simulink model "hopper_6dof_NED_v3_fluid_integration"  (R2026a)
settings: Solver=FixedStepAuto  StopTime=30  FixedStep=1e-3  RelTol=1e-5
InitFcn:
  | load('FuelPropsData.mat');
undefined symbols (not defined in the file): bp, cg_init, dcg_dMfu_table, dcg_dMox_table, dI_dMfu_table, dI_dMox_table, ENGINE, engine_cg, engine_mass, fu_masses, g, IN, K1flat, K2grid, MoI_init, mount_cg, OUT, ox_masses, pressureLevels, r_leg_1, r_leg_2, r_leg_3, r_leg_4, tank_r, TANKS, Target_Trajectory_full, tbl1, tbl2, tgrid, unom, uwndTable, VEH, vwndTable
libraries: fl_lib x43, nesl_utility x31, matrix_library x18, SimscapeFluids_lib x13, simulink_extras x7, slpidlib x7, simulink x7, dspindex x3, sl_discontinuities x2, aerolibanim x1, commrandsrc3 x1, aerolibutil x1
(part 2 of 7)

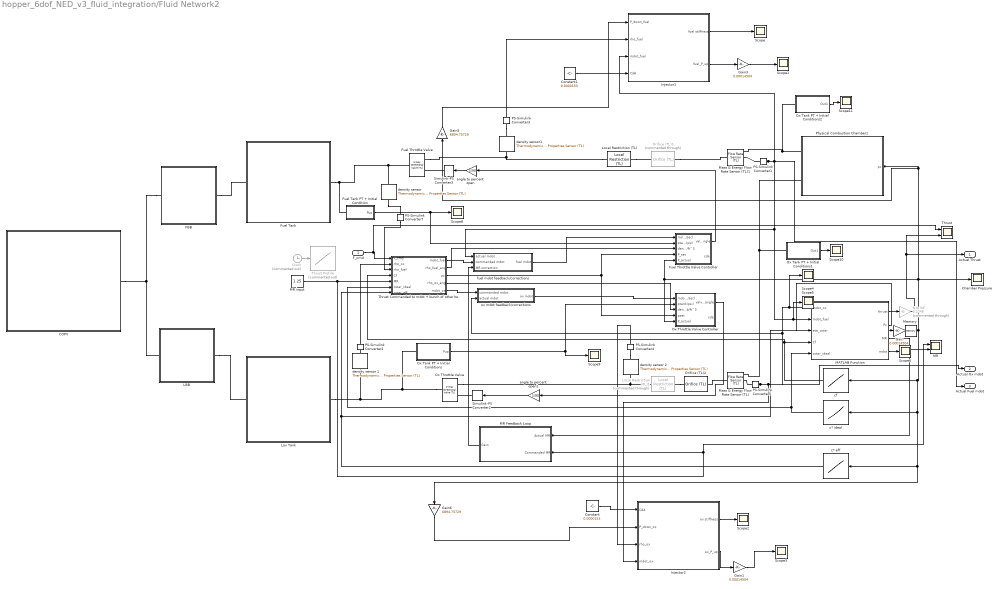
== system hopper_6dof_NED_v3_fluid_integration/Fluid Network2 ==
  F_cmd : Inport
  COPV : Subsystem
  Chamber Pressure : Scope
      settings: ActiveDisplayYMinimum=24.4768520913143  ActiveDisplayYMaximum=276.14956071215624  DataLoggingVariableName=ScopeData22
  Clock : Clock  Commented=on
  Constant : Constant  Value=0.0000153
  Constant1 : Constant  Value=0.0000153
  FBB : Subsystem
  Fuel Tank : Subsystem
  Fuel Tank PT + Initial Condition : Subsystem
  Fuel Throttle Valve : SimscapeFluids_lib/Thermal Liquid/Valves & Orifices/Directional Control Valves/2-Way Directional Valve (TL)  valve_spec=fluids.thermal_liquid.valves.directional_control_valves.enum.ValveSpec.Table1DAreaOpening  S_max=1 m  del_S_max=5e-3 m  area_max=1e-4 m^2  area_leak=1e-10 m^2  del_S_TLU=[0 0.3 0.4 0.5 0.6 0.7 0.8 0.9 1.0] m  valve_area_TLU=[1e-9 1.7065e-07 1.0239e-06 3.5836e-06 7.8498e-06 1.4164e-05 2.3038e-05 3.4812e-05 5.0000e-05] m^2  del_S_flow_TLU=[0, .002, .004, .007, .017] m  p_diff_TLU=[.3, .5, .7] MPa  vol_flow_TLU=1e-3 * [1.7e-05, 2e-05, 2.6e-05; .0035, .0045, .0053; .7, .9, 1.06; 1.96, 2.5, 3; 6, 7.7, 9.13] m^3/s  mdot_TLU=[1.7e-05, 2e-05, 2.6e-05; .0035, .0045, .0053; .7, .9, 1.06; 1.96, 2.5, 3; 6, 7.7, 9.13] kg/s  T_ref_in=293.15 K  p_ref_in=0.101325 MPa  Cd=1  Re_c=150  smoothing_factor=0.01  pressure_recovery=false  area=0.01 m^2
  Fuel Throttle Valve Controller : Subsystem
  Gain : Gain  Gain=0.00014504
  Gain1 : Gain  Gain=0.00014504
  Gain3 : Gain  Gain=0.00014504
  Gain5 : Gain  Gain=6894.75729
  Gain6 : Gain  Gain=6894.75729
  Injector1 : Subsystem
  Injector2 : Subsystem
  LBB : Subsystem
  Local Restriction (TL) : fl_lib/Thermal Liquid/Elements/Local Restriction (TL)  restriction_type=foundation.enum.restriction_type.fixed  restriction_area=0.0000153 m^2  min_area=1e-10 m^2  max_area=0.005 m^2  area=0.000153 m^2  Cd=1  Re_c=150  pressure_recovery=true
  Local Restriction (TL)1 : fl_lib/Thermal Liquid/Elements/Local Restriction (TL)  Commented=through  restriction_type=foundation.enum.restriction_type.fixed  restriction_area=0.0000153 m^2  min_area=1e-10 m^2  max_area=0.005 m^2  area=0.000153 m^2  Cd=1  Re_c=150  pressure_recovery=true
  Lox Tank : Subsystem
  MATLAB Function : MATLAB Function  TreatAsAtomicUnit=on
  MR : Scope  NumInputPorts=2
      settings: ActiveDisplayYMinimum=0.081947452963374467  ActiveDisplayYMaximum=2.5817499803566988
  MR Feedback Loop : Subsystem
  MR input : Constant  Value=1.25
  Mass & Energy Flow Rate Sensor (TL) : fl_lib/Thermal Liquid/Sensors/Flow Rate Sensor (TL)  mass_flow_measure=true  volumetric_flow_measure=false  energy_flow_measure=true
  Mass & Energy Flow Rate Sensor (TL)1 : fl_lib/Thermal Liquid/Sensors/Flow Rate Sensor (TL)  mass_flow_measure=true  volumetric_flow_measure=false  energy_flow_measure=true
  Memory : Memory  InitialCondition=300
  N to lbf : Gain  Commented=through  Gain=0.2248
  Orifice (TL)1 : SimscapeFluids_lib/Thermal Liquid/Valves & Orifices/Orifice (TL)  Commented=through  orifice_type=foundation.enum.constant_variable.constant  constant_orifice_spec=fluids.thermal_liquid.valves.enum.ConstantOrificeSpec.Area  variable_orifice_spec=fluids.thermal_liquid.valves.enum.orifice_spec.linear  orifice_area_constant=0.0000153 m^2  p_diff_TLU_constant=[-4, -3, -2, -1, -.5, 0, .5, 1, 2, 3, 4] MPa  vol_flow_TLU_constant=[-2.44, -2.12, -1.68, -1.22, -.84, 0, .85, 1.21, 1.7, 2.09, 2.41] .* 1e-3 m^3/s  mdot_TLU_constant=[-2.44, -2.12, -1.68, -1.22, -.84, 0, .85, 1.21, 1.7, 2.09, 2.41] kg/s  S_min=0 m  del_S=5e-3 m  open_orientation=fluids.thermal_liquid.valves.enum.orifice_orientation.positive  area_max=1e-4 m^2  area_leak=1e-10 m^2  S_TLU=[0, .002, .004, .007, .017] m  orifice_area_TLU=[1e-09, 2.0352e-07, 4.0736e-05, .00011438, .00034356] m^2  Cd=1  Re_c=150  smoothing_factor=0.01  pressure_recovery=false  S_flow_TLU=[0, .002, .004, .007, .017] m  p_diff_TLU=[.3, .5, .7] MPa  vol_flow_TLU=1e-3 * [1.7e-05, 2e-05, 2.6e-05; .0035, .0045, .0053; .7, .9, 1.06; 1.96, 2.5, 3; 6, 7.7, 9.13] m^3/s  mdot_TLU=[1.7e-05, 2e-05, 2.6e-05; .0035, .0045, .0053; .7, .9, 1.06; 1.96, 2.5, 3; 6, 7.7, 9.13] kg/s  T_ref_in=293.15 K  p_ref_in=0.101325 MPa  area=0.01 m^2
  Orifice (TL)2 : SimscapeFluids_lib/Thermal Liquid/Valves & Orifices/Orifice (TL)  orifice_type=foundation.enum.constant_variable.constant  constant_orifice_spec=fluids.thermal_liquid.valves.enum.ConstantOrificeSpec.Area  variable_orifice_spec=fluids.thermal_liquid.valves.enum.orifice_spec.linear  orifice_area_constant=0.0000153 m^2  p_diff_TLU_constant=[-4, -3, -2, -1, -.5, 0, .5, 1, 2, 3, 4] MPa  vol_flow_TLU_constant=[-2.44, -2.12, -1.68, -1.22, -.84, 0, .85, 1.21, 1.7, 2.09, 2.41] .* 1e-3 m^3/s  mdot_TLU_constant=[-2.44, -2.12, -1.68, -1.22, -.84, 0, .85, 1.21, 1.7, 2.09, 2.41] kg/s  S_min=0 m  del_S=5e-3 m  open_orientation=fluids.thermal_liquid.valves.enum.orifice_orientation.positive  area_max=1e-4 m^2  area_leak=1e-10 m^2  S_TLU=[0, .002, .004, .007, .017] m  orifice_area_TLU=[1e-09, 2.0352e-07, 4.0736e-05, .00011438, .00034356] m^2  Cd=1  Re_c=150  smoothing_factor=0.01  pressure_recovery=false  S_flow_TLU=[0, .002, .004, .007, .017] m  p_diff_TLU=[.3, .5, .7] MPa  vol_flow_TLU=1e-3 * [1.7e-05, 2e-05, 2.6e-05; .0035, .0045, .0053; .7, .9, 1.06; 1.96, 2.5, 3; 6, 7.7, 9.13] m^3/s  mdot_TLU=[1.7e-05, 2e-05, 2.6e-05; .0035, .0045, .0053; .7, .9, 1.06; 1.96, 2.5, 3; 6, 7.7, 9.13] kg/s  T_ref_in=293.15 K  p_ref_in=0.101325 MPa  area=0.01 m^2
  Ox Tank PT + Initial Conditions : Subsystem
  Ox Tank PT + Initial Conditions1 : Subsystem
  Ox Tank PT + Initial Conditions2 : Subsystem
  Ox Throttle Valve : SimscapeFluids_lib/Thermal Liquid/Valves & Orifices/Directional Control Valves/2-Way Directional Valve (TL)  valve_spec=fluids.thermal_liquid.valves.directional_control_valves.enum.ValveSpec.Table1DAreaOpening  S_max=1 m  del_S_max=5e-3 m  area_max=1e-4 m^2  area_leak=1e-10 m^2  del_S_TLU=[0 0.3 0.4 0.5 0.6 0.7 0.8 0.9 1.0] m  valve_area_TLU=[1e-9 1.7065e-07 1.0239e-06 3.5836e-06 7.8498e-06 1.4164e-05 2.3038e-05 3.4812e-05 5.0000e-05] m^2  del_S_flow_TLU=[0, .002, .004, .007, .017] m  p_diff_TLU=[.3, .5, .7] MPa  vol_flow_TLU=1e-3 * [1.7e-05, 2e-05, 2.6e-05; .0035, .0045, .0053; .7, .9, 1.06; 1.96, 2.5, 3; 6, 7.7, 9.13] m^3/s  mdot_TLU=[1.7e-05, 2e-05, 2.6e-05; .0035, .0045, .0053; .7, .9, 1.06; 1.96, 2.5, 3; 6, 7.7, 9.13] kg/s  T_ref_in=293.15 K  p_ref_in=0.101325 MPa  Cd=1  Re_c=150  smoothing_factor=0.01  pressure_recovery=false  area=0.01 m^2
  Ox Throttle Valve Controller : Subsystem
  PS-Simulink Converter{1..5,7} (6 alike) : nesl_utility/PS-Simulink Converter  PhysicalDomain=network_engine_domain  SubClassName=ps_output  LeftPortType=input  RightPortType=output  PseudoPeriodic=off  Frequencies=[]  VectorFormat=inherit  Unit=inherit  AffineConversion=off
  Physical Combustion Chamber1 : Subsystem
  Scope{,1..6,8..11} (11 alike) : Scope
      Scope settings: ActiveDisplayYMinimum=-0.024254245068718681  ActiveDisplayYMaximum=0.21828827495285463  DataLoggingVariableName=ScopeData40
      Scope1 settings: ActiveDisplayYMinimum=-37.465424615708343  ActiveDisplayYMaximum=337.50135970832162  DataLoggingVariableName=ScopeData42
      Scope10 settings: ActiveDisplayYMinimum=-62.731329785992315  ActiveDisplayYMaximum=586.85713455527571  DataLoggingVariableName=ScopeData51
      Scope11 settings: ActiveDisplayYMinimum=-62.499971643181283  ActiveDisplayYMaximum=562.49999684924239  DataLoggingVariableName=ScopeData52
      Scope2 settings: ActiveDisplayYMinimum=-0.025857157768165939  ActiveDisplayYMaximum=0.4462125176132366  DataLoggingVariableName=ScopeData43
      Scope3 settings: ActiveDisplayYMinimum=-1  ActiveDisplayYMaximum=1  DataLoggingVariableName=ScopeData44
      Scope4 settings: ActiveDisplayYMinimum=-0.071595374751251564  ActiveDisplayYMaximum=0.64519605918641931  DataLoggingVariableName=ScopeData53
      Scope5 settings: ActiveDisplayYMinimum=-0.05515719954820638  ActiveDisplayYMaximum=0.49713967255882957  DataLoggingVariableName=ScopeData54
      Scope6 settings: ActiveDisplayYMinimum=-0.1205205125313115  ActiveDisplayYMaximum=1.086247175831931  DataLoggingVariableName=ScopeData55
      Scope8 settings: ActiveDisplayYMinimum=481.05362935967628  ActiveDisplayYMaximum=536.06057249536832  DataLoggingVariableName=ScopeData49
      Scope9 settings: ActiveDisplayYMinimum=492.10107740407369  ActiveDisplayYMaximum=524.51908611925091  DataLoggingVariableName=ScopeData50
  Simulink-PS Converter2 : nesl_utility/Simulink-PS Converter  PhysicalDomain=network_engine_domain  SubClassName=ps_input  LeftPortType=input  RightPortType=output  PseudoPeriodic=off  Frequencies=[]  NoiseDistribution=none  NoiseParameters=[]  Unit=1  AffineConversion=off  FilteringAndDerivatives=filter  SimscapeFilterOrder=1  InputFilterTimeConstant=0.001  UdotUserProvided=0
  Simulink-PS Converter3 : nesl_utility/Simulink-PS Converter  PhysicalDomain=network_engine_domain  SubClassName=ps_input  LeftPortType=input  RightPortType=output  PseudoPeriodic=off  Frequencies=[]  NoiseDistribution=none  NoiseParameters=[]  Unit=1  AffineConversion=off  FilteringAndDerivatives=filter  SimscapeFilterOrder=1  InputFilterTimeConstant=0.001  UdotUserProvided=0
  Thrust : Scope  NumInputPorts=2
      settings: ActiveDisplayYMinimum=-215.53569406218494  ActiveDisplayYMaximum=1942.1553478833205  DataLoggingVariableName=ScopeData21
  Thrust Commanded to mdot + bunch of other bs : MATLAB Function  TreatAsAtomicUnit=on
  Thrust Profile : Lookup_n-D  Commented=on  NumberOfTableDimensions=1  BreakpointsForDimension1=|  Table=|  InternalRulePriority=Speed  RndMeth=Simplest
      BreakpointsForDimension1=|
      | [0
      | 2.46e-15
      | 4.93e-15
      | 1.31e-14
      | 1.85798e-4
      | 3.71595e-4
      | 1.300583e-3
      | 5.945524e-3
      | 2.917023e-2
      | 1.452937e-1
      | 3.251823e-1
      | 6.176896e-1
      | 1.048884
      | 1.648122
      | 2.452841
      | 3.452841
      | 4.452841
      | 5.452841
      | 6.452841
      | 7.452841
      | 8.452841
      | 9.452841
      | 10.45284
      | 11.45284
      | 12.45284
      | 13.45284
      | 14.45284
      | 15.45284
      | 16.26888
      | 17.26888
      | 18.26888
      | 19.26888
      | 20.26888
      | 21.26888
      | 21.82014
      | 22.37140
      | 23.10183
      | 24.10183
      | 25.10183
      | 26.10183
      | 27.10183
      | 28.10183
      | 29.10183
      | 29.70287]
      Table=|
      | [1115.929794
      | 1115.929794
      | 1115.929794
      | 1115.929794
      | 1116.015031
      | 1116.100248
      | 1116.526042
      | 1118.647732
      | 1129.075722
      | 1176.888468
      | 1237.984070
      | 1309.087819
      | 1365.657208
      | 1382.500173
      | 1347.869214
      | 1276.732855
      | 1209.886660
      | 1007.359221
      | 890.000000
      | 890.000000
      | 890.000000
      | 890.000000
      | 970.372958
      | 1015.368113
      | 1034.720854
      | 1040.888013
      | 1040.596927
      | 896.870767
      | 890.000000
      | 890.000000
      | 890.000000
      | 890.000000
      | 890.000000
      | 890.000000
      | 1074.062231
      | 1213.486737
      | 1218.338865
      | 1172.384789
      | 1114.978943
      | 1066.195681
      | 1030.043331
      | 1004.841448
      | 987.599936
      | 979.912878]
  angle to percent open : Gain  Gain=1/90
  angle to percent open1 : Gain  Gain=1/90
  c* eff : Lookup_n-D  NumberOfTableDimensions=1  BreakpointsForDimension1=[125 295]  Table=[0.8 0.85]  InternalRulePriority=Speed  RndMeth=Simplest
  c* ideal : Lookup_n-D  NumberOfTableDimensions=1  BreakpointsForDimension1=[100 110 120 130 140 150 160 170 180 190 200 210 220 230 240 250 260 270 280 290 300 310 320 330 340 350]  Table=[1492.810749 1492.812678 1492.815823 1492.820080 1492.825344 1492.831574 1492.838703 1492.846662 1492.855462 1492.865052 1492.875406 1492.886504 1492.898325 1492.910854 1492.924078 1492.937982 1492.952558 1492.967791 1492.983688 1493.000184 1493.017345 1493.035113 1493.053494 1493.072480 1493.092063 1493.112237]  InternalRulePriority=Speed  RndMeth=Simplest
  cf : Lookup_n-D  NumberOfTableDimensions=1  BreakpointsForDimension1=[125 295]  Table=[1.42 1.57]  InternalRulePriority=Speed  RndMeth=Simplest
  density sensor : fl_lib/Thermal Liquid/Sensors/Thermodynamic Properties Sensor (TL)  internal_energy=false  density=true  specific_heat=false
  density sensor 1 : fl_lib/Thermal Liquid/Sensors/Thermodynamic Properties Sensor (TL)  internal_energy=false  density=true  specific_heat=false
  density sensor 2 : fl_lib/Thermal Liquid/Sensors/Thermodynamic Properties Sensor (TL)  internal_energy=false  density=true  specific_heat=false
  density sensor1 : fl_lib/Thermal Liquid/Sensors/Thermodynamic Properties Sensor (TL)  internal_energy=false  density=true  specific_heat=false
  fuel mdot feedback/corrections : Subsystem
  ox mdot feedback/corrections : Subsystem
  Actual Thrust : Outport
  Actual Ox mdot : Outport  Port=2
  Actual Fuel mdot : Outport  Port=3
  wires:
  MATLAB Function/4(mdot) -> Scope6/1
  PS-Simulink Converter4/1 -> Injector2/3(rho_ox)
  PS-Simulink Converter3/1 -> Injector1/2(rho_fuel)
  Memory/1 -> Chamber Pressure/1, Fuel Throttle Valve Controller/5(P_actual), Ox Throttle Valve Controller/5(P_actual), Physical Combustion Chamber1/1(pc), Gain5/1, cf/1, c* ideal/1, c* eff/1, Gain6/1
  Gain6/1 -> Injector2/2(P_down_ox)
  Gain5/1 -> Injector1/1(P_down_fuel)
  Gain1/1 -> Scope3/1
  Gain3/1 -> Scope1/1
  Ox Tank PT + Initial Conditions2/1(Out1) -> Scope11/1
  Ox Tank PT + Initial Conditions1/1(Out1) -> Scope10/1
  PS-Simulink Converter7/1 -> Thrust Commanded to mdot + bunch of other bs/3(rho_fuel)
  Constant1/1 -> Injector1/4(CdA)
  Constant/1 -> Injector2/1(CdA)
  Injector2/2(ox_P_up) -> Gain1/1
  Injector2/1(ox stiffness) -> Scope2/1
  Injector1/2(fuel_P_up) -> Gain3/1
  Injector1/1(fuel stiffness) -> Scope/1
  PS-Simulink Converter1/1 -> fuel mdot feedback/corrections/1(actual mdot), MATLAB Function/2(mdot_fuel), Scope5/1, Injector1/3(mdot_fuel), Actual Fuel mdot/1
  PS-Simulink Converter5/1 -> ox mdot feedback/corrections/2(actual mdot), MATLAB Function/1(mdot_ox), Scope4/1, Injector2/4(mdot_ox), Actual Ox mdot/1
  F_cmd/1 -> Thrust Commanded to mdot + bunch of other bs/1(F_cmd), Thrust/1
  cf/1 -> MATLAB Function/4(Cf), Thrust Commanded to mdot + bunch of other bs/4(Cf)
  c* eff/1 -> MATLAB Function/3(eta_cstar), Thrust Commanded to mdot + bunch of other bs/7(cstar_eff)
  PS-Simulink Converter2/1 -> Thrust Commanded to mdot + bunch of other bs/2(rho_ox)
  Thrust Commanded to mdot + bunch of other bs/3(pc) -> Fuel Throttle Valve Controller/4(P_set), Ox Throttle Valve Controller/4(pset)
  MR input/1 -> Thrust Commanded to mdot + bunch of other bs/5(MR), MR/1, MR Feedback Loop/2(Commanded MR)
  MR Feedback Loop/1(Gain) -> fuel mdot feedback/corrections/3(MR correction)
  ox mdot feedback/corrections/1(ox mdot) -> Ox Throttle Valve Controller/1(mdot (lb/sec))
  MATLAB Function/2(Pc) -> Gain/1
  Fuel Throttle Valve Controller/1(valve angle) -> angle to percent open/1
  Gain/1 -> Memory/1
  MATLAB Function/1(thrust) -> N to lbf/1
  Clock/1 -> Thrust Profile/1
  Thrust Commanded to mdot + bunch of other bs/4(rho_ox_eng) -> Ox Throttle Valve Controller/3(density lb/ft^3)
  Thrust Commanded to mdot + bunch of other bs/5(mdot_ox) -> ox mdot feedback/corrections/1(commanded mdot)
  fuel mdot feedback/corrections/1(fuel mdot) -> Fuel Throttle Valve Controller/1(mdot (lb/sec))
  MATLAB Function/3(MR) -> MR/2, MR Feedback Loop/1(Actual MR)
  angle to percent open1/1 -> Simulink-PS Converter2/1
  angle to percent open/1 -> Simulink-PS Converter3/1
  Ox Tank PT + Initial Conditions/1(Pup) -> Ox Throttle Valve Controller/2(ptank(psi)), Scope9/1
  Thrust Commanded to mdot + bunch of other bs/1(mdot_fuel) -> fuel mdot feedback/corrections/2(commanded mdot)
  N to lbf/1 -> Actual Thrust/1, Thrust/2
  Fuel Tank PT + Initial Condition/1(Pup) -> Fuel Throttle Valve Controller/2(ptank(psi)), Scope8/1
  Thrust Commanded to mdot + bunch of other bs/2(rho_fuel_eng) -> Fuel Throttle Valve Controller/3(density lb/ft^3)
  Ox Throttle Valve Controller/1(valve angle) -> angle to percent open1/1
  c* ideal/1 -> Thrust Commanded to mdot + bunch of other bs/6(cstar_ideal), MATLAB Function/5(cstar_ideal)
  connections:
  Local Restriction (TL)1/RConn1 -- Orifice (TL)2/LConn1
  Local Restriction (TL)/RConn1 -- Orifice (TL)1/LConn1
  PS-Simulink Converter4/LConn1 -- density sensor 2/RConn1
  PS-Simulink Converter3/LConn1 -- density sensor1/RConn1
  Orifice (TL)2/RConn1 -- Mass & Energy Flow Rate Sensor (TL)/LConn1
  Orifice (TL)1/RConn1 -- Mass & Energy Flow Rate Sensor (TL)1/LConn1
  Local Restriction (TL)/LConn1 -- density sensor1/LConn1 -- Fuel Throttle Valve/RConn2
  Simulink-PS Converter2/RConn1 -- Ox Throttle Valve/RConn1
  PS-Simulink Converter1/LConn1 -- Mass & Energy Flow Rate Sensor (TL)1/RConn2
  FBB/LConn1 -- LBB/LConn1 -- COPV/RConn1
  Ox Throttle Valve/LConn1 -- Ox Tank PT + Initial Conditions/LConn1 -- density sensor 1/LConn1 -- Lox Tank/RConn1
  density sensor/RConn1 -- PS-Simulink Converter7/LConn1
  Mass & Energy Flow Rate Sensor (TL)/RConn1 -- Physical Combustion Chamber1/RConn2 -- Ox Tank PT + Initial Conditions1/LConn1
  FBB/RConn1 -- Fuel Tank/LConn1
  Ox Tank PT + Initial Conditions2/LConn1 -- Physical Combustion Chamber1/RConn1 -- Mass & Energy Flow Rate Sensor (TL)1/RConn1
  density sensor 2/LConn1 -- Local Restriction (TL)1/LConn1 -- Ox Throttle Valve/RConn2
  PS-Simulink Converter5/LConn1 -- Mass & Energy Flow Rate Sensor (TL)/RConn2
  Simulink-PS Converter3/RConn1 -- Fuel Throttle Valve/RConn1
  Fuel Tank PT + Initial Condition/LConn1 -- density sensor/LConn1 -- Fuel Throttle Valve/LConn1 -- Fuel Tank/RConn1
  LBB/RConn1 -- Lox Tank/LConn1
  density sensor 1/RConn1 -- PS-Simulink Converter2/LConn1

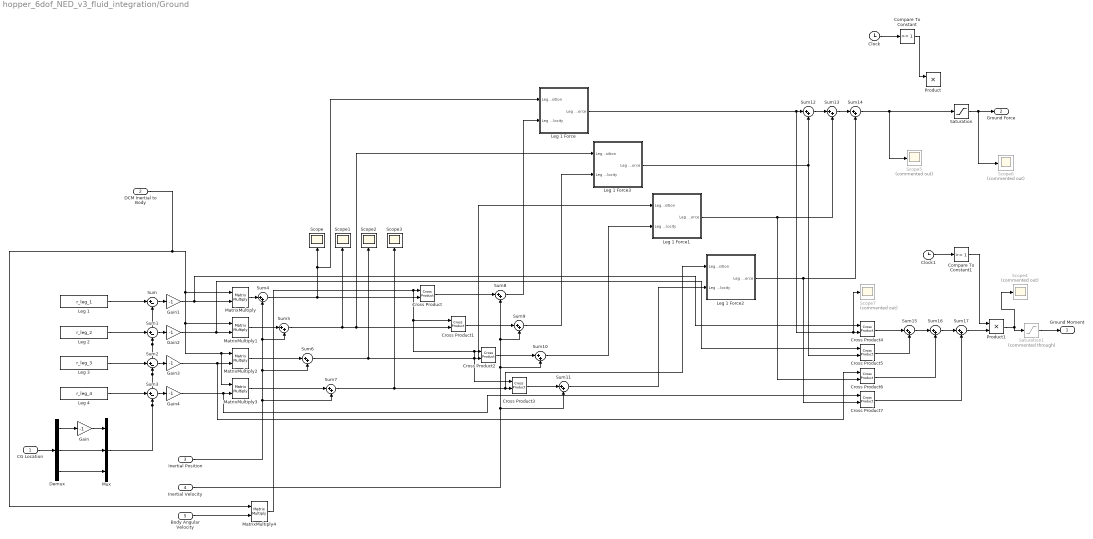
== system hopper_6dof_NED_v3_fluid_integration/Ground  ==
  CG Location : Inport
  DCM Inertial to Body : Inport  Port=2
  Inertial Position : Inport  Port=3
  Inertial Velocity : Inport  Port=4
  Body Angular Velocity : Inport  Port=5
  Clock : Clock
  Clock1 : Clock
  Compare To Constant : simulink/Logic and Bit Operations/Compare To Constant  relop=>=  const=1  OutDataTypeStr=boolean
  Compare To Constant1 : simulink/Logic and Bit Operations/Compare To Constant  relop=>=  const=1  OutDataTypeStr=boolean
  Cross Product{,1..7} (8 alike) : matrix_library/Cross Product
  Demux : Demux  Outputs=3
  Gain{,1..4} (5 alike) : Gain  Gain=-1
  Leg 1 : Constant  Value=r_leg_1
  Leg 1 Force : Subsystem
  Leg 1 Force1 : Subsystem
  Leg 1 Force2 : Subsystem
  Leg 1 Force3 : Subsystem
  Leg 2 : Constant  Value=r_leg_2
  Leg 3 : Constant  Value=r_leg_3
  Leg 4 : Constant  Value=r_leg_4
  MatrixMultiply{,1..4} (5 alike) : Product  Multiplication=Matrix(*)
  Mux : Mux  Inputs=3
  Product : Product
  Product1 : Product
  Saturation : Saturate  UpperLimit=inf  LowerLimit=0
  Saturation1 : Saturate  Commented=through  UpperLimit=inf  LowerLimit=0
  Scope{,1..3} (4 alike) : Scope
      Scope settings: ActiveDisplayYMinimum=-19.811154048207108  ActiveDisplayYMaximum=167.31101950999761  DataLoggingVariableName=ScopeData24
      Scope1 settings: ActiveDisplayYMinimum=182.10765195211306  ActiveDisplayYMaximum=183.93696889205802  DataLoggingVariableName=ScopeData30
      Scope2 settings: DataLoggingVariableName=ScopeData31
      Scope3 settings: DataLoggingVariableName=ScopeData42
  Scope{4..7} (4 alike) : Scope  Commented=on
      Scope4 settings: ActiveDisplayYMinimum=-3.0293963365637429E+7  ActiveDisplayYMaximum=2.2731893212350109E+8  DataLoggingVariableName=ScopeData43
      Scope5 settings: ActiveDisplayYMinimum=-31343.151613259419  ActiveDisplayYMaximum=282088.36451933486  DataLoggingVariableName=ScopeData44
      Scope6 settings: ActiveDisplayYMinimum=-136.62925150266653  ActiveDisplayYMaximum=1229.6632635239991  DataLoggingVariableName=ScopeData45
      Scope7 settings: ActiveDisplayYMinimum=-3.5823523450793636E+8  ActiveDisplayYMaximum=5.8466661508525646E+8  DataLoggingVariableName=ScopeData61
  Sum{,1..3} (4 alike) : Sum  Inputs=|+-
  Sum{4..17} (14 alike) : Sum  Inputs=|++
  Ground Moment : Outport
  Ground Force : Outport  Port=2
  wires:
  Demux/2 -> Mux/2
  Demux/3 -> Mux/3
  Leg 1/1 -> Sum/1
  Leg 2/1 -> Sum1/1
  Leg 3/1 -> Sum2/1
  Leg 4/1 -> Sum3/1
  Mux/1 -> Sum3/2, Sum1/2, Sum/2, Sum2/2
  Sum/1 -> Gain1/1
  DCM Inertial to Body/1 -> MatrixMultiply4/1, MatrixMultiply1/1, MatrixMultiply3/1, MatrixMultiply2/1, MatrixMultiply/1
  Sum1/1 -> Gain2/1
  Sum2/1 -> Gain3/1
  Sum3/1 -> Gain4/1
  MatrixMultiply3/1 -> Sum7/1
  MatrixMultiply2/1 -> Sum6/1
  MatrixMultiply1/1 -> Sum5/1
  MatrixMultiply/1 -> Sum4/1
  Inertial Position/1 -> Sum7/2, Sum6/2, Sum5/2, Sum4/2
  Sum4/1 -> Scope/1, Leg 1 Force/1(Leg Position), Cross Product/2
  Sum5/1 -> Leg 1 Force3/1(Leg Position), Cross Product1/2, Scope1/1
  Sum6/1 -> Leg 1 Force1/1(Leg Position), Cross Product2/2, Scope2/1
  Sum7/1 -> Leg 1 Force2/1(Leg Position), Cross Product3/2, Scope3/1
  Body Angular Velocity/1 -> MatrixMultiply4/2
  MatrixMultiply4/1 -> Cross Product1/1, Cross Product3/1, Cross Product2/1, Cross Product/1
  Cross Product/1 -> Sum8/1
  Cross Product1/1 -> Sum9/1
  Cross Product2/1 -> Sum10/1
  Cross Product3/1 -> Sum11/1
  Inertial Velocity/1 -> Sum11/2, Sum10/2, Sum9/2, Sum8/2
  Leg 1 Force/1(Leg 1 Force) -> Scope7/1, Cross Product4/2, Sum12/1
  Leg 1 Force3/1(Leg 1 Force) -> Cross Product5/2, Sum12/2
  Sum12/1 -> Sum13/1
  Leg 1 Force1/1(Leg 1 Force) -> Cross Product6/2, Sum13/2
  Sum13/1 -> Sum14/1
  Leg 1 Force2/1(Leg 1 Force) -> Cross Product7/2, Sum14/2
  Cross Product4/1 -> Sum15/1
  Sum15/1 -> Sum16/1
  Cross Product5/1 -> Sum15/2
  Cross Product6/1 -> Sum16/2
  Sum16/1 -> Sum17/1
  Cross Product7/1 -> Sum17/2
  Sum8/1 -> Leg 1 Force/2(Leg Velocity)
  Sum9/1 -> Leg 1 Force3/2(Leg Velocity)
  Sum10/1 -> Leg 1 Force1/2(Leg Velocity)
  Sum11/1 -> Leg 1 Force2/2(Leg Velocity)
  Saturation/1 -> Ground Force/1, Scope6/1
  Saturation1/1 -> Ground Moment/1
  Gain/1 -> Mux/1
  Gain1/1 -> Cross Product4/1, MatrixMultiply/2
  Gain2/1 -> Cross Product5/1, MatrixMultiply1/2
  Gain3/1 -> Cross Product6/1, MatrixMultiply2/2
  Gain4/1 -> Cross Product7/1, MatrixMultiply3/2
  Sum14/1 -> Saturation/1, Scope5/1
  Clock1/1 -> Compare To Constant1/1
  Compare To Constant1/1 -> Product1/1
  Sum17/1 -> Product1/2
  Product1/1 -> Scope4/1, Saturation1/1
  CG Location/1 -> Demux/1
  Demux/1 -> Gain/1
  Clock/1 -> Compare To Constant/1
  Compare To Constant/1 -> Product/1

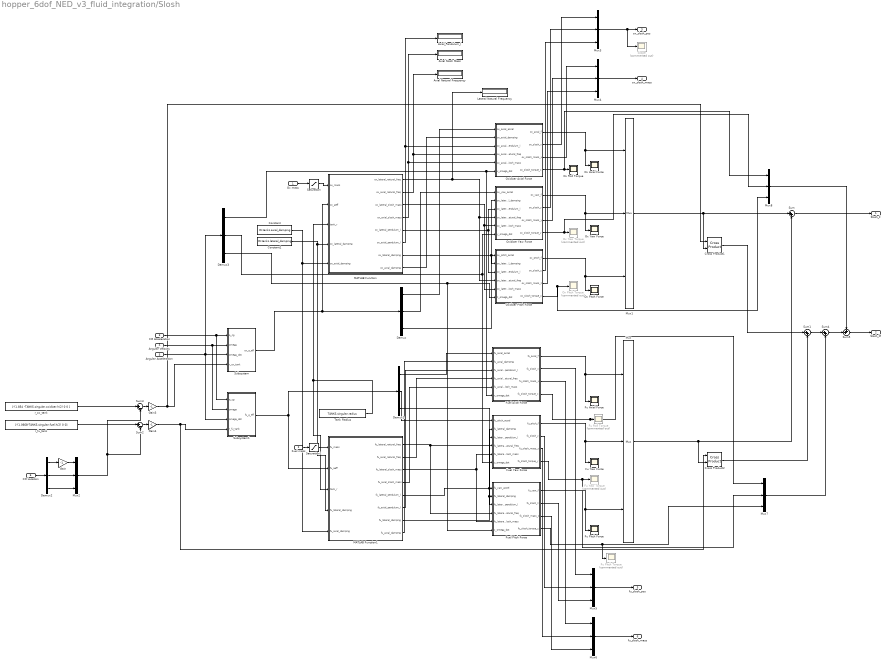
== system hopper_6dof_NED_v3_fluid_integration/Slosh ==
  Ox mass : Inport
  Fuel mass : Inport  Port=2
  CG Acceleration : Inport  Port=3
  Angular Velocity : Inport  Port=4
  Angular Acceleration : Inport  Port=5
  CG Location : Inport  Port=6
  Axial Natural Frequency : Display
  Axial Slosh Mass : Display
  Axial_Pendulum_l : Display
  Constant : Constant  Value=IN.tanks.axial_damping
  Constant1 : Constant  Value=IN.tanks.lateral_damping
  Cross Product1 : matrix_library/Cross Product
  Cross Product2 : matrix_library/Cross Product
  Demux{,1..3} (4 alike) : Demux  Outputs=3
  Fu Axial Force : Scope
      settings: ActiveDisplayYMinimum=-4.5487995330933861  ActiveDisplayYMaximum=10.430303988696288  DataLoggingVariableName=ScopeData38
  Fu Pitch Force : Scope
      settings: ActiveDisplayYMinimum=-49.446700881181073  ActiveDisplayYMaximum=52.013559841067675  DataLoggingVariableName=ScopeData40
  Fu Pitch Torque : Scope  Commented=on
      settings: ActiveDisplayYMinimum=-0.19116574787256713  ActiveDisplayYMaximum=0.19970427620804132  DataLoggingVariableName=ScopeData87
  Fu Roll Torque : Scope  Commented=on
      settings: ActiveDisplayYMinimum=-9.5580450498277436  ActiveDisplayYMaximum=8.6061310713641461  DataLoggingVariableName=ScopeData86
  Fu Yaw Force : Scope
      settings: ActiveDisplayYMinimum=-33.187691556065026  ActiveDisplayYMaximum=34.918104624839692  DataLoggingVariableName=ScopeData39
  Fu Yaw Torque : Scope  Commented=on
      settings: ActiveDisplayYMinimum=-3.6886267521568623  ActiveDisplayYMaximum=3.9647425854021145  DataLoggingVariableName=ScopeData82
  Fuel Axial Force : Subsystem
  Fuel Pitch Force : Subsystem
  Fuel Yaw Force : Subsystem
  Gain : Gain  Gain=-1
  Gain3 : Gain  Gain=-1
  Gain4 : Gain  Gain=-1
  Lateral Natural Frequency : Display
  MATLAB Function : MATLAB Function  TreatAsAtomicUnit=on
  MATLAB Function1 : MATLAB Function  TreatAsAtomicUnit=on
  Mux{,1..8} (9 alike) : Mux  Inputs=3
  Ox Axial Force : Scope
      settings: ActiveDisplayYMinimum=-3.9139633032684662  ActiveDisplayYMaximum=18.1052993336341  DataLoggingVariableName=ScopeData34
  Ox Pitch Force : Scope
      settings: ActiveDisplayYMinimum=-3.7836149976681615  ActiveDisplayYMaximum=11.014640697122998  DataLoggingVariableName=ScopeData36
  Ox Pitch Torque : Scope  Commented=on
      settings: ActiveDisplayYMinimum=-0.69593653498138675  ActiveDisplayYMaximum=0.79680864639954685  DataLoggingVariableName=ScopeData85
  Ox Roll Torque : Scope
      settings: ActiveDisplayYMinimum=-0.15656949128956149  ActiveDisplayYMaximum=0.79158034254760723  DataLoggingVariableName=ScopeData80
  Ox Yaw Force : Scope
      settings: ActiveDisplayYMinimum=-23.507612676925252  ActiveDisplayYMaximum=5.0177421078517668  DataLoggingVariableName=ScopeData37
  Ox Yaw Torque : Scope  Commented=on
      settings: ActiveDisplayYMinimum=-0.3482323750211066  ActiveDisplayYMaximum=0.31743853430357161  DataLoggingVariableName=ScopeData81
  Oxidizer Axial Force : Subsystem
  Oxidizer Pitch Force : Subsystem
  Oxidizer Yaw Force : Subsystem
  Saturation : Saturate  UpperLimit=inf  LowerLimit=0.01
  Saturation1 : Saturate  UpperLimit=inf  LowerLimit=0.01
  Scope : Scope  Commented=on
      settings: ActiveDisplayYMinimum=-0.0849364779794028  ActiveDisplayYMaximum=0.368207880424993  DataLoggingVariableName=ScopeData35
  Subsystem : Subsystem
  Subsystem1 : Subsystem
  Sum : Sum  Inputs=|++
  Sum1 : Sum  Inputs=|++
  Sum2 : Sum  Inputs=|+-
  Sum3 : Sum  Inputs=|+-
  Sum4 : Sum  Inputs=|++
  Sum5 : Sum  Inputs=++|
  Tank Radius : Constant  Value=TANKS.singular.radius  SampleTime=-1
  r_fu_tank : Constant  Value=[-(1.0668-TANKS.singular.fuel.h/2) 0 0]
  r_ox_tank : Constant  Value=[-(1.854 -TANKS.singular.oxidizer.h/2) 0 0 ]
  Slosh_F : Outport
  Slosh_M : Outport  Port=2
  ox_slosh_pos : Outport  Port=3
  ox_slosh_mass : Outport  Port=4
  fu_slosh_pos : Outport  Port=5
  fu_slosh_mass : Outport  Port=6
  wires:
  Ox mass/1 -> Saturation/1
  CG Acceleration/1 -> Subsystem/1(a_cg), Subsystem1/1(a_cg)
  Angular Velocity/1 -> Subsystem/2(omega), Subsystem1/2(omega)
  Angular Acceleration/1 -> Subsystem/3(omega_dot), Subsystem1/3(omega_dot), Demux3/1
  Fuel mass/1 -> Saturation1/1
  Subsystem/1(ox_a_eff) -> Demux/1, MATLAB Function/2(ox_aeff)
  Subsystem1/1(fu_a_eff) -> Demux1/1, MATLAB Function1/2(fu_aeff)
  Demux/1 -> Oxidizer Axial Force/1(ox_axial_accel)
  Demux/2 -> Oxidizer Yaw Force/1(ox_yaw_accel)
  Demux/3 -> Oxidizer Pitch Force/1(ox_pitch_accel)
  Demux1/1 -> Fuel Axial Force/1(fu_axial_accel)
  Demux1/2 -> Fuel Yaw Force/1(fu_pitch_accel)
  Demux1/3 -> Fuel Pitch Force/1(fu_yaw_accel)
  MATLAB Function/1(ox_lateral_natural_freq) -> Lateral Natural Frequency/1, Oxidizer Pitch Force/4(ox_lateral_natural_freq), Oxidizer Yaw Force/4(ox_lateral_natural_freq)
  MATLAB Function/2(ox_axial_natural_freq) -> Axial Natural Frequency/1, Oxidizer Axial Force/4(ox_axial_natural_freq)
  MATLAB Function/3(ox_lateral_slosh_mass) -> Oxidizer Pitch Force/5(ox_lateral_slosh_mass), Oxidizer Yaw Force/5(ox_lateral_slosh_mass)
  MATLAB Function/4(ox_axial_slosh_mass) -> Axial Slosh Mass/1, Oxidizer Axial Force/5(ox_axial_slosh_mass)
  MATLAB Function/5(ox_lateral_pendulum_l) -> Oxidizer Yaw Force/3(ox_lateral_pendulum_l), Oxidizer Pitch Force/3(ox_lateral_pendulum_l)
  MATLAB Function/6(ox_axial_pendulum_l) -> Axial_Pendulum_l/1, Oxidizer Axial Force/3(ox_axial_pendulum_l)
  MATLAB Function/7(ox_lateral_damping) -> Oxidizer Yaw Force/2(ox_lateral_damping), Oxidizer Pitch Force/2(ox_lateral_damping)
  MATLAB Function/8(ox_axial_damping) -> Oxidizer Axial Force/2(ox_axial_damping)
  MATLAB Function1/1(fu_lateral_natural_freq) -> Fuel Pitch Force/4(fu_lateral_natural_freq), Fuel Yaw Force/4(fu_lateral_natural_freq)
  MATLAB Function1/2(fu_axial_natural_freq) -> Fuel Axial Force/4(fu_axial_natural_freq)
  MATLAB Function1/3(fu_lateral_slosh_mass) -> Fuel Yaw Force/5(fu_lateral_slosh_mass), Fuel Pitch Force/5(fu_lateral_slosh_mass)
  MATLAB Function1/4(fu_axial_slosh_mass) -> Fuel Axial Force/5(fu_axial_slosh_mass)
  MATLAB Function1/5(fu_lateral_pendulum_l) -> Fuel Yaw Force/3(fu_lateral_pendulum_l), Fuel Pitch Force/3(fu_lateral_pendulum_l)
  MATLAB Function1/6(fu_axial_pendulum_l) -> Fuel Axial Force/3(fu_axial_pendulum_l)
  MATLAB Function1/7(fu_lateral_damping) -> Fuel Yaw Force/2(fu_lateral_damping), Fuel Pitch Force/2(fu_lateral_damping)
  MATLAB Function1/8(fu_axial_damping) -> Fuel Axial Force/2(fu_axial_damping)
  Fuel Axial Force/1(fu_axial_f) -> Fu Axial Force/1, Mux/1
  Fuel Yaw Force/1(fu_pitch_f) -> Fu Yaw Force/1, Mux/2
  Oxidizer Axial Force/1(ox_axial_f) -> Ox Axial Force/1, Mux1/1
  Oxidizer Yaw Force/1(ox_yaw_f) -> Ox Yaw Force/1, Mux1/2
  Mux1/1 -> Cross Product1/2, Sum/1
  Mux/1 -> Sum/2, Cross Product2/2
  Sum/1 -> Slosh_F/1
  Cross Product1/1 -> Sum1/1
  Cross Product2/1 -> Sum1/2
  Tank Radius/1 -> MATLAB Function1/3(tank_r), MATLAB Function/3(tank_r)
  r_ox_tank/1 -> Sum3/1
  r_fu_tank/1 -> Sum2/1
  Mux2/1 -> Sum2/2, Sum3/2
  Sum3/1 -> Gain3/1
  Sum2/1 -> Gain4/1
  Constant/1 -> MATLAB Function/5("ox_axial_damping "), MATLAB Function1/5("fu_axial_damping ")
  Constant1/1 -> MATLAB Function/4("ox_lateral_damping "), MATLAB Function1/4("fu_lateral_damping ")
  Fuel Pitch Force/1(fu_yaw_f) -> Mux/3, Fu Pitch Force/1
  Oxidizer Pitch Force/1(ox_pitch_f) -> Mux1/3, Ox Pitch Force/1
  Gain3/1 -> Cross Product1/1, Subsystem/4(r_ox_tank)
  Gain4/1 -> Cross Product2/1, Subsystem1/4(r_fu_tank)
  Demux2/3 -> Mux2/3
  CG Location/1 -> Demux2/1
  Demux2/2 -> Mux2/2
  Demux2/1 -> Gain/1
  Gain/1 -> Mux2/1
  Oxidizer Yaw Force/2(ox_slosh_y) -> Mux3/2
  Mux3/1 -> Scope/1, ox_slosh_pos/1
  Oxidizer Axial Force/3(ox_slosh_mass_x) -> Mux4/1
  Oxidizer Yaw Force/3(ox_slosh_mass_y) -> Mux4/2
  Oxidizer Pitch Force/2(ox_slosh_z) -> Mux3/3
  Oxidizer Pitch Force/3(ox_slosh_mass_z) -> Mux4/3
  Mux4/1 -> ox_slosh_mass/1
  Mux5/1 -> fu_slosh_pos/1
  Mux6/1 -> fu_slosh_mass/1
  Fuel Yaw Force/2(fu_slosh_y) -> Mux5/2
  Fuel Pitch Force/2(fu_slosh_z) -> Mux5/3
  Fuel Axial Force/3(fu_slosh_mass_x) -> Mux6/1
  Fuel Yaw Force/3(fu_slosh_mass_y) -> Mux6/2
  Fuel Pitch Force/3(fu_slosh_mass_z) -> Mux6/3
  Oxidizer Axial Force/2(ox_slosh_x) -> Mux3/1
  Fuel Axial Force/2(fu_slosh_x) -> Mux5/1
  Demux3/1 -> Oxidizer Axial Force/6(x_omega_dot), Fuel Axial Force/6(x_omega_dot)
  Demux3/2 -> Fuel Yaw Force/6(y_omega_dot), Oxidizer Yaw Force/6(y_omega_dot)
  Demux3/3 -> Fuel Pitch Force/6(z_omega_dot), Oxidizer Pitch Force/6(z_omega_dot)
  Fuel Axial Force/4(fu_slosh_torque_x) -> Mux7/1, Fu Roll Torque/1
  Fuel Yaw Force/4(fu_slosh_torque_y) -> Mux7/2, Fu Yaw Torque/1
  Fuel Pitch Force/4(fu_slosh_torque_z) -> Mux7/3, Fu Pitch Torque/1
  Oxidizer Axial Force/4(ox_slosh_torque_x) -> Mux8/1, Ox Roll Torque/1
  Oxidizer Pitch Force/4(ox_slosh_torque_z) -> Ox Pitch Torque/1, Mux8/3
  Sum1/1 -> Sum4/1
  Sum5/1 -> Slosh_M/1
  Sum4/1 -> Sum5/2
  Oxidizer Yaw Force/4(ox_slosh_torque_y) -> Mux8/2, Ox Yaw Torque/1
  Mux8/1 -> Sum5/1
  Mux7/1 -> Sum4/2
  Saturation/1 -> MATLAB Function/1(ox_mass)
  Saturation1/1 -> MATLAB Function1/1(fu_mass)

== system hopper_6dof_NED_v3_fluid_integration/Subsystem ==
  Thrust : Inport
  Fuel mdot : Lookup_n-D  NumberOfTableDimensions=1  BreakpointsForDimension1=bp  Table=tbl1  InternalRulePriority=Speed  RndMeth=Simplest
  Ox mdot : Lookup_n-D  NumberOfTableDimensions=1  BreakpointsForDimension1=bp  Table=tbl2  InternalRulePriority=Speed  RndMeth=Simplest
  Fu_mdot : Outport
  Ox_mdot : Outport  Port=2
  wires:
  Thrust/1 -> Ox mdot/1, Fuel mdot/1
  Fuel mdot/1 -> Fu_mdot/1
  Ox mdot/1 -> Ox_mdot/1

== system hopper_6dof_NED_v3_fluid_integration/Subsystem1 ==
  Ox_mdot : Inport
  Fu_mdot : Inport  Port=2
  Integrator : Integrator
  Integrator1 : Integrator
  Ox Mass1 : Constant  Value=IN.propulsion.oxidizer_mass
  Ox Mass2 : Constant  Value=IN.propulsion.fuel_mass
  Saturation : Saturate  UpperLimit=IN.propulsion.oxidizer_mass  LowerLimit=0
  Saturation1 : Saturate  UpperLimit=IN.propulsion.fuel_mass  LowerLimit=0
  Sum : Sum  Inputs=|-+
  Sum1 : Sum  Inputs=|-+
  Ox Mass : Outport
  Fuel Mass : Outport  Port=2
  wires:
  Ox_mdot/1 -> Integrator/1
  Integrator/1 -> Sum/1
  Ox Mass1/1 -> Sum/2
  Sum/1 -> Saturation/1
  Saturation/1 -> Ox Mass/1
  Sum1/1 -> Saturation1/1
  Saturation1/1 -> Fuel Mass/1
  Fu_mdot/1 -> Integrator1/1
  Ox Mass2/1 -> Sum1/2
  Integrator1/1 -> Sum1/1

== system hopper_6dof_NED_v3_fluid_integration/Subsystem2 ==
  Thrust : Inport
  Ox mass : Inport  Port=2
  Fu mass : Inport  Port=3
  If : If  NumInputs=2  IfExpression=u1 > 0 & u2 > 0
  If Action Subsystem : Subsystem  TreatAsAtomicUnit=on
  If Action Subsystem1 : Subsystem  TreatAsAtomicUnit=on
  Merge : Merge
  "Thrust " : Outport
  wires:
  Ox mass/1 -> If/1
  Fu mass/1 -> If/2
  If/1 -> If Action Subsystem/Action
  If/2 -> If Action Subsystem1/Action
  Thrust/1 -> If Action Subsystem1/1(Thrust), If Action Subsystem/1(Thrust)
  If Action Subsystem/1(Out1) -> Merge/1
  If Action Subsystem1/1(Out1) -> Merge/2
  Merge/1 -> "Thrust "/1

== system hopper_6dof_NED_v3_fluid_integration/Subsystem3 ==
  Z : Inport
  W : Inport  Port=2
  Clock : Clock
  Compare To Constant : simulink/Logic and Bit Operations/Compare To Constant  relop=>=  const=5  OutDataTypeStr=boolean
  Constant : Constant
  If : If  NumInputs=2  IfExpression=u1 > -1e-3 & u2 > 0
  If Action Subsystem : Subsystem  TreatAsAtomicUnit=on
  Product : Product
  wires:
  Z/1 -> If/1
  W/1 -> If/2
  If/1 -> If Action Subsystem/Action
  Clock/1 -> Compare To Constant/1
  Compare To Constant/1 -> Product/2
  Constant/1 -> Product/1
  Product/1 -> If Action Subsystem/1(In1)

== system hopper_6dof_NED_v3_fluid_integration/Subsystem4 ==
  Thrust : Inport
  Position : Inport  Port=2
  Velocity : Inport  Port=3
  Demux : Demux  Outputs=3
  Demux1 : Demux  Outputs=3
  If : If  NumInputs=2  IfExpression=u1 > -0.05 & u2 > 0
  If Action Subsystem : Subsystem  TreatAsAtomicUnit=on
  If Action Subsystem1 : Subsystem  TreatAsAtomicUnit=on
  Merge : Merge
  "Thrust " : Outport
  wires:
  If Action Subsystem1/1(Out1) -> Merge/2
  Merge/1 -> "Thrust "/1
  If Action Subsystem/1(Out1) -> Merge/1
  Thrust/1 -> If Action Subsystem1/1(Thrust), If Action Subsystem/1(Thrust)
  Position/1 -> Demux/1
  Demux1/3 -> If/2
  Demux/3 -> If/1
  If/1 -> If Action Subsystem1/Action
  If/2 -> If Action Subsystem/Action
  Velocity/1 -> Demux1/1

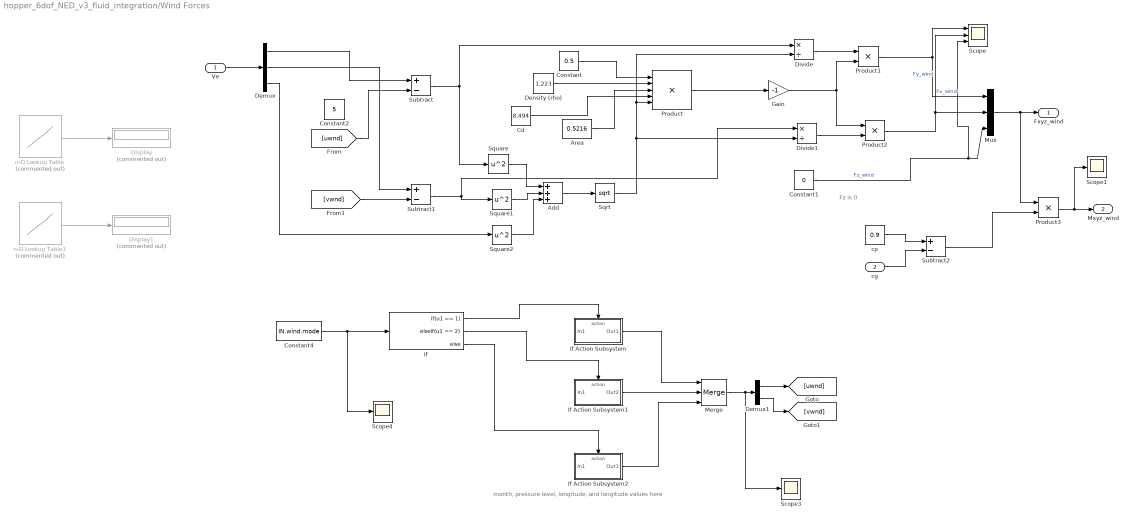
== system hopper_6dof_NED_v3_fluid_integration/Wind Forces ==
  note: month, pressure level, longitude, and longitude values here
  note: Fz is 0
  Ve : Inport
  cg : Inport  Port=2
  Add : Sum  Inputs=+++
  Area : Constant  Value=0.5216
  Cd : Constant  Value=8.494
  Constant : Constant  Value=0.5
  Constant1 : Constant  Value=0
  Constant2 : Constant  Value=5
  Constant4 : Constant  Value=IN.wind.mode
  Demux : Demux  Outputs=3
  Demux1 : Demux  Outputs=2
  Density (rho) : Constant  Value=1.223
  Display : Display  Commented=on
  Display1 : Display  Commented=on
  Divide : Product  Inputs=*/
  Divide1 : Product  Inputs=*/
  Gain : Gain  Gain=-1
  If : If  IfExpression=u1 == 1  ElseIfExpressions=u1 == 2
  If Action Subsystem : Subsystem  TreatAsAtomicUnit=on
  If Action Subsystem1 : Subsystem  TreatAsAtomicUnit=on
  If Action Subsystem2 : Subsystem  TreatAsAtomicUnit=on
  Merge : Merge  Inputs=3
  Mux : Mux  Inputs=3
  Product : Product  Inputs=5
  Product1 : Product
  Product2 : Product
  Product3 : Product
  Scope : Scope  NumInputPorts=3
      settings: ActiveDisplayYMinimum=-3.3865408119999993  ActiveDisplayYMaximum=30.478867308  DataLoggingVariableName=ScopeData58
  Scope1 : Scope
      settings: ActiveDisplayYMinimum=-7.3042803283540865  ActiveDisplayYMaximum=15.553528390525987  DataLoggingVariableName=ScopeData89
  Scope3 : Scope
      settings: ActiveDisplayYMinimum=1  ActiveDisplayYMaximum=3  DataLoggingVariableName=ScopeData90
  Scope4 : Scope
      settings: ActiveDisplayYMinimum=1  ActiveDisplayYMaximum=3  DataLoggingVariableName=ScopeData91
  Sqrt : Sqrt
  Square : Math  Operator=square
  Square1 : Math  Operator=square
  Square2 : Math  Operator=square
  Subtract : Sum  Inputs=+-
  Subtract1 : Sum  Inputs=+-
  Subtract2 : Sum  Inputs=+-
  cp : Constant  Value=0.9
  n-D Lookup Table : Lookup_n-D  Commented=on  NumberOfTableDimensions=4  BreakpointsForDimension1=1:12  BreakpointsForDimension2=pressureLevels  BreakpointsForDimension3=[32.5 35]  BreakpointsForDimension4=[82.5 85]  Table=uwndTable  ExtrapMethod=Clip  InternalRulePriority=Speed  RndMeth=Simplest
      settings: InputPortMap=u0,u1,u2,u3
  n-D Lookup Table1 : Lookup_n-D  Commented=on  NumberOfTableDimensions=4  BreakpointsForDimension1=1:12  BreakpointsForDimension2=pressureLevels  BreakpointsForDimension3=[32.5 35]  BreakpointsForDimension4=[82.5 85]  Table=vwndTable  InternalRulePriority=Speed  RndMeth=Simplest
      settings: InputPortMap=u0,u1,u2,u3
  Fxyz_wind : Outport
  Mxyz_wind : Outport  Port=2
  wires:
  If/1 -> If Action Subsystem/Action
  Mux/1 -> Product3/1, Fxyz_wind/1
  [vwnd] -> Subtract1/2
  n-D Lookup Table1/1 -> Display1/1
  Demux/3 -> Square2/1
  cp/1 -> Subtract2/1
  Divide1/1 -> Product2/2
  Square/1 -> Add/1
  Merge/1 -> Scope3/1, Demux1/1
  Demux1/2 -> [vwnd]
  Product3/1 -> Scope1/1, Mxyz_wind/1
  Gain/1 -> Product1/2, Product2/1
  Subtract2/1 -> Product3/2
  Ve/1 -> Demux/1
  Subtract/1 -> Divide/1, Square/1
  If/2 -> If Action Subsystem1/Action
  Sqrt/1 -> Divide1/2, Divide/2, Product/5
  Demux1/1 -> [uwnd]
  [uwnd] -> Subtract/2
  Area/1 -> Product/3
  Square2/1 -> Add/3
  Product2/1 -> Scope/2, Mux/2  "Fy_wind"
  Constant4/1 -> Scope4/1, If/1
  Constant1/1 -> Scope/3, Mux/3  "Fz_wind"
  If/3 -> If Action Subsystem2/Action
  Product1/1 -> Scope/1, Mux/1  "Fx_wind"
  Cd/1 -> Product/4
  Subtract1/1 -> Square1/1, Divide1/1
  Density (rho)/1 -> Product/2
  If Action Subsystem/1(Out1) -> Merge/1
  cg/1 -> Subtract2/2
  If Action Subsystem2/1(Out1) -> Merge/3
  Constant/1 -> Product/1
  n-D Lookup Table/1 -> Display/1
  Demux/2 -> Subtract1/1
  If Action Subsystem1/1(Out2) -> Merge/2
  Divide/1 -> Product1/1
  Add/1 -> Sqrt/1
  Product/1 -> Gain/1
  Square1/1 -> Add/2
  Demux/1 -> Subtract/1

== system hopper_6dof_NED_v3_fluid_integration/Control Inputs -> Fxyz & Mxyz/EDF Dynamics ==
  Cmd Torque : Inport
  Divide : Product  Inputs=*/
  Product : Product
  Product1 : Product
  Quantizer2 : Quantizer  QuantizationInterval=IN.rcs.resolution
  Radius : Constant  Value=TANKS.singular.radius
  Rate Limiter : RateLimiter  RisingSlewLimit=25  FallingSlewLimit=-25  SampleTimeMode=inherited
  Saturation : Saturate  Commented=through  UpperLimit=1  LowerLimit=0  ZeroCross=off
  Saturation1 : Saturate  UpperLimit=IN.rcs.max_thrust  LowerLimit=-IN.rcs.max_thrust  ZeroCross=off
  Transfer Fcn : TransferFcn  Denominator=[IN.rcs_time_constant 1]
  max Thrust : Constant  Value=IN.rcs.max_thrust
  "Real Torque " : Outport
  wires:
  Divide/1 -> Saturation/1
  Radius/1 -> Product/2
  Product/1 -> Product1/2, Divide/2
  Cmd Torque/1 -> Divide/1
  max Thrust/1 -> Product/1
  Transfer Fcn/1 -> Product1/1
  Product1/1 -> Quantizer2/1
  Saturation/1 -> Transfer Fcn/1
  Quantizer2/1 -> Rate Limiter/1
  Rate Limiter/1 -> Saturation1/1
  Saturation1/1 -> "Real Torque "/1
